simulink model "afe_inv_ttype_psm"  (R2026a)
settings: Solver=ode23tb  StopTime=simlength  FixedStep=tc  MaxStep=glb_time.tc
values from neighbouring files (symbols this model uses):
  afe_ctrl = ctrl_afe_setup(glb_time.ts_afe, grid_emu.omega_grid_nom)    [init_model.m]
  afe_pwm_phase_shift_mod1 = 0    [init_model.m]
  DThs_init = 0    [init_model.m]
  filters = setup_global_filters(glb_time.ts_afe, glb_time.ts_inv, glb_time.ts_dab, glb_time.tc)    [init_model.m]
  frt_data = frt_settings(test_index, test_subindex, asymmetric_error_type,      enable_frt_1, enable_frt_2, start_time_LVRT, deepPOSxi, deepPOSeta, deepNEGxi, deepNEGeta)    [init_model.m]
  glb_time = timing_setup(fpwm_afe, trgo_afe, fpwm_inv, trgo_inv, fpwm_single_phase_inv, trgo_single_phase_inv, fpwm_dab, trgo_dab,      fpwm_psfbc, trgo_psfbc, fpwm_isop_rail, trgo_isop_rail, fpwm_cllc, trgo_cllc, t_measure, tc_factor, tc_decimation, delay_pwm, dead_time_afe,      dead_time_inv, dead_time_single_phase_inv, dead_time_dab, dead_time_psfbc, dead_time_isop_rail, dead_time_cllc)    [init_model.m]
  grid_emu = grid_three_phase_emulator('Dyn11', delta_star, grid_nominal_power, application_voltage, us1, us2, fgrid,                  eq_grid_inductance, eq_grid_resistance, eta, ucc, i1m, p_iron, n1, n2, core_area, core_length, mur,                  up_xi_pu_ref, up_eta_pu_ref, un_xi_pu_ref, un_eta_pu_ref)    [init_model.m]
  i_react_pos_ref_2 = -ixi_ref_mod1*tan(acos(0.95))    [init_model.m]
  i_react_pos_ref_3 = ixi_ref_mod1*tan(acos(0.95))    [init_model.m]
  ixi_ref_mod1 = -0.85    [init_model.m]
  ki_align = 18    [init_model.m]
  kp_align = 0.25    [init_model.m]
  lim_down_align = -0.05    [init_model.m]
  lim_up_align = 0.05    [init_model.m]
  mavarage_filter_frequency_base_order = 2    [init_model.m]
  omega_m_sim = psm.omega_m_bez    [init_model.m]
  psm = psm_calculus()    [init_model.m]
  psm_ctrl = ctrl_pmsm_setup(glb_time.ts_inv, psm.omega_bez, u_psm_scale, psm.Jm_norm)    [init_model.m]
  simlength = 1.75    [init_model.m]
  Tambient = 40    [init_model.m]
  time_aux_power_supply_fault = 1e3    (= 1000)    [init_model.m]
  time_gain_afe_module_1 = 1.0002    [init_model.m]
  time_gain_inv_module_2 = 1.001    [init_model.m]
  time_i_react_pos_ref_1 = start_time_LVRT + error_length + 0.335    [init_model.m]
  time_i_react_pos_ref_2 = time_i_react_pos_ref_1 + 0.5    (= 0.5)    [init_model.m]
  time_start_motor_control = 0.25    [init_model.m]
  torque_overload_factor = 1    [init_model.m]
  u_cm_comp_mod1 = 0    [init_model.m]
  u_psm_scale_ekf = sqrt(3)/2 * 2/3 * hwdata.inv.udc_nom/psm.ubez    [init_model.m]
undefined symbols (not defined in the file or in its folder): hwdata, magnitude, omega_m_bez, rpm_base, torque_base
libraries: fl_lib x74, nesl_utility x43, moving_average_filter x10, moving_average_filter_cc x8, discrete_time_low_pass_filter x4, sl_discontinuities x3, single_phase_transformer_lib x3, linear_double_integrator_observer_ccaller x2, threephase_inductor_lib x2, dclink_for_three_levels x2, three_phase_three_level_ttype_inverter_ideal_switch_based_model x2, cstblocks_lti x2
(part 2 of 9)

== system afe_inv_ttype_psm/global timing/time_afe3 ==
  Gain : Gain  Gain=k
  time_1 : Clock
  Out1 : Outport
  wires:
  Gain/1 -> Out1/1
  time_1/1 -> Gain/1

== system afe_inv_ttype_psm/global timing/time_inv1 ==
  correction_time : Inport
  Constant : Constant
  Gain : Gain  Gain=k
  Product : Product
  Sum : Sum  Inputs=|++
  time_1 : Clock
  Out1 : Outport
  wires:
  time_1/1 -> Gain/1
  Gain/1 -> Product/1
  Product/1 -> Out1/1
  correction_time/1 -> Sum/1
  Constant/1 -> Sum/2
  Sum/1 -> Product/2

== system afe_inv_ttype_psm/grid/grid_emulator ==
  3ph_Dyg : Subsystem
  Bus Selector : BusSelector  OutputSignals=ua_grid_emu,ub_grid_emu,uc_grid_emu
  Bus Selector1 : BusSelector  OutputSignals=gamma_grid_emulator,omega_grid_emulator
  Controlled Voltage Source : fl_lib/Electrical/Electrical Sources/Controlled Voltage Source
  Controlled Voltage Source1 : fl_lib/Electrical/Electrical Sources/Controlled Voltage Source
  Controlled Voltage Source2 : fl_lib/Electrical/Electrical Sources/Controlled Voltage Source
  Electrical Reference : fl_lib/Electrical/Electrical Elements/Electrical Reference
  Simulink-PS Converter : nesl_utility/Simulink-PS Converter  PhysicalDomain=network_engine_domain  SubClassName=ps_input  LeftPortType=input  RightPortType=output  PseudoPeriodic=off  Frequencies=[]  NoiseDistribution=none  NoiseParameters=[]  Unit=V  AffineConversion=on  FilteringAndDerivatives=provide  SimscapeFilterOrder=1  InputFilterTimeConstant=0.001  UdotUserProvided=0
  Simulink-PS Converter1 : nesl_utility/Simulink-PS Converter  PhysicalDomain=network_engine_domain  SubClassName=ps_input  LeftPortType=input  RightPortType=output  PseudoPeriodic=off  Frequencies=[]  NoiseDistribution=none  NoiseParameters=[]  Unit=V  AffineConversion=on  FilteringAndDerivatives=provide  SimscapeFilterOrder=1  InputFilterTimeConstant=0.001  UdotUserProvided=0
  Simulink-PS Converter2 : nesl_utility/Simulink-PS Converter  PhysicalDomain=network_engine_domain  SubClassName=ps_input  LeftPortType=input  RightPortType=output  PseudoPeriodic=off  Frequencies=[]  NoiseDistribution=none  NoiseParameters=[]  Unit=V  AffineConversion=on  FilteringAndDerivatives=provide  SimscapeFilterOrder=1  InputFilterTimeConstant=0.001  UdotUserProvided=0
  Solver Configuration : nesl_utility/Solver Configuration  PhysicalDomain=network_engine_domain  SubClassName=solver  LeftPortType=input  RightPortType=generic  Tones=[]  Harmonics=[]  SimulateNoise=off  Profile=off  UseLocalSampling=off  EnableSwitchedLinearOptims=on  FrequencyDomain=off  UseCCode=off  RelTol=0.001  AbsTol=0.001  MinStep=1e-09  ToWorkspace=off  RevertToSquareIcSolve=off  NumHomotopyIterations=100  PhasorMode=off  PhasorModeNumHarmonics=1  ConsistencySolver=NEWTON_FTOL  CanonicalOrdering=UNORDERED  OptimizeIntermediates=UNOPTIMIZED  IndexReductionMethod=DerivativeReplacement  DoDC=on  ResidualTolerance=1e-09  ConsistencyTolSource=GLOBAL  ConsistencyAbsTol=0.001  ConsistencyRelTol=0.001  ConsistencyTolFactor=0.001  UseLocalSolver=on  LocalSolverChoice=NE_BACKWARD_EULER_ADVANCER  ResolveIndetEquations=on  FunctionEvalNumThread=1  LocalSolverSampleTime=glb_time.tc  DoFixedCost=on  MaxNonlinIter=nonlinear_iterations  MaxModeIter=2  ComputeImpulses=off  ImpulseIterations=2  LinearAlgebra=auto  LinearAlgebraNumThread=0  EquationFormulation=NE_TIME_EF  DelaysMemoryBudget=1024  AutomaticFiltering=on  FilteringTimeConstant=0.001  PartitionStorageMethod=AS_NEEDED  PartitionMemoryBudget=1024  PartitionMethod=ROBUST  MultibodyUseLocalSolver=off  MultibodyLocalSolverChoice=ODE1  MultibodyLocalSolverSampleTime=0.001
  three_phase_voltage_source_with_frt_emulator : three_phase_voltage_with_frt_emulator/three_phase_voltage_source_with_frt_emulator  nominal_frequency_m=grid_emu.fgrid_nom  nominal_voltage_m=grid_emu.us_primary_nom  Vemu_ref_norm_m=grid_emu.Vemu_ref_norm  vp_xi_pu_m=grid_emu.up_xi_pu_ref  vp_eta_pu_m=grid_emu.up_eta_pu_ref  vn_xi_pu_m=grid_emu.un_xi_pu_ref  vn_eta_pu_m=grid_emu.un_eta_pu_ref  Am=filters.afe.SOF_50Hz.ss_c.A  Bm=filters.afe.SOF_50Hz.ss_c.B  Cm=filters.afe.SOF_50Hz.ss_c.C  enable_frt_1_m=frt_data.enable_frt_1  enable_frt_2_m=frt_data.enable_frt_2  start_time_LVRT_m=frt_data.start_time_LVRT  end_time_LVRT_m=frt_data.end_time_LVRT  deepPOSxi_m=frt_data.deepPOSxi  deepPOSeta_m=frt_data.deepPOSeta  deepNEGxi_m=frt_data.deepNEGxi  deepNEGeta_m=frt_data.deepNEGeta  Amplitude_U_m=frt_data.Amplitude_U  Amplitude_V_m=frt_data.Amplitude_V  Amplitude_W_m=frt_data.Amplitude_W  t_ramp_m=frt_data.t_ramp  Phase_shift_m=frt_data.Phase_shift
  threephase_vi_measures : Subsystem
  u1 : PMIOPort  Side=Right
  u2 : PMIOPort  Port=2  Side=Right
  u3 : PMIOPort  Port=3  Side=Right
  tag scope: gamma_grid_emulator=global, omega_grid_emulator=global
  wires:
  Bus Selector1/2 -> [omega_grid_emulator]  "<omega_grid_emulator>"
  Bus Selector1/1 -> [gamma_grid_emulator]  "<gamma_grid_emulator>"
  Bus Selector/2 -> Simulink-PS Converter1/1  "<ub_grid_emu>"
  Bus Selector/3 -> Simulink-PS Converter2/1  "<uc_grid_emu>"
  three_phase_voltage_source_with_frt_emulator/1 -> Bus Selector1/1, Bus Selector/1
  Bus Selector/1 -> Simulink-PS Converter/1  "<ua_grid_emu>"
  connections:
  Simulink-PS Converter/RConn1 -- Controlled Voltage Source/RConn1
  Simulink-PS Converter1/RConn1 -- Controlled Voltage Source1/RConn1
  Simulink-PS Converter2/RConn1 -- Controlled Voltage Source2/RConn1
  Electrical Reference/LConn1 -- Controlled Voltage Source/RConn2 -- Controlled Voltage Source1/RConn2 -- Controlled Voltage Source2/RConn2 -- Solver Configuration/RConn1
  3ph_Dyg/RConn1 -- u1/RConn1
  3ph_Dyg/RConn2 -- u2/RConn1
  3ph_Dyg/RConn3 -- u3/RConn1
  3ph_Dyg/LConn1 -- threephase_vi_measures/RConn1
  3ph_Dyg/LConn2 -- threephase_vi_measures/RConn2
  3ph_Dyg/LConn3 -- threephase_vi_measures/RConn3
  Controlled Voltage Source/LConn1 -- threephase_vi_measures/LConn1
  Controlled Voltage Source1/LConn1 -- threephase_vi_measures/LConn2
  Controlled Voltage Source2/LConn1 -- threephase_vi_measures/LConn3

== system afe_inv_ttype_psm/grid/threephase_vi_measures ==
  Bus Creator : BusCreator  Inputs=6
  Current Sensor : fl_lib/Electrical/Electrical Sensors/Current Sensor
  Current Sensor1 : fl_lib/Electrical/Electrical Sensors/Current Sensor
  Current Sensor2 : fl_lib/Electrical/Electrical Sensors/Current Sensor
  Electrical Reference1 : fl_lib/Electrical/Electrical Elements/Electrical Reference
  Selector : Selector  InputPortWidth=6  IndexOptions=Index vector (dialog)  Indices=[1 2 3]  OutputSizes=1
  Selector1 : Selector  InputPortWidth=6  IndexOptions=Index vector (dialog)  Indices=[4 5 6]  OutputSizes=1
  Voltage Sensor : fl_lib/Electrical/Electrical Sensors/Voltage Sensor
  Voltage Sensor1 : fl_lib/Electrical/Electrical Sensors/Voltage Sensor
  Voltage Sensor2 : fl_lib/Electrical/Electrical Sensors/Voltage Sensor
  ia_grid : nesl_utility/PS-Simulink Converter  PhysicalDomain=network_engine_domain  SubClassName=ps_output  LeftPortType=input  RightPortType=output  PseudoPeriodic=off  Frequencies=[]  VectorFormat=1-D array  Unit=A  AffineConversion=off
  ib_grid : nesl_utility/PS-Simulink Converter  PhysicalDomain=network_engine_domain  SubClassName=ps_output  LeftPortType=input  RightPortType=output  PseudoPeriodic=off  Frequencies=[]  VectorFormat=1-D array  Unit=A  AffineConversion=off
  ic_grid : nesl_utility/PS-Simulink Converter  PhysicalDomain=network_engine_domain  SubClassName=ps_output  LeftPortType=input  RightPortType=output  PseudoPeriodic=off  Frequencies=[]  VectorFormat=1-D array  Unit=A  AffineConversion=off
  ig_abc/ug_abc : Scope  NumInputPorts=2
      settings: SampleTime=glb_time.tc  ActiveDisplayYMinimum=-662.618491750231  ActiveDisplayYMaximum=662.00821995187164  DataLoggingVariableName=ScopeData2
  ua_grid : nesl_utility/PS-Simulink Converter  PhysicalDomain=network_engine_domain  SubClassName=ps_output  LeftPortType=input  RightPortType=output  PseudoPeriodic=off  Frequencies=[]  VectorFormat=1-D array  Unit=V  AffineConversion=off
  ub_grid : nesl_utility/PS-Simulink Converter  PhysicalDomain=network_engine_domain  SubClassName=ps_output  LeftPortType=input  RightPortType=output  PseudoPeriodic=off  Frequencies=[]  VectorFormat=1-D array  Unit=V  AffineConversion=off
  uc_grid : nesl_utility/PS-Simulink Converter  PhysicalDomain=network_engine_domain  SubClassName=ps_output  LeftPortType=input  RightPortType=output  PseudoPeriodic=off  Frequencies=[]  VectorFormat=1-D array  Unit=V  AffineConversion=off
  Ua : PMIOPort  Side=Left
  ua : PMIOPort  Port=2  Side=Right
  Ub : PMIOPort  Port=3  Side=Left
  ub : PMIOPort  Port=4  Side=Right
  Uc : PMIOPort  Port=5  Side=Left
  uc : PMIOPort  Port=6  Side=Right
  tag scope: ig_abc=global, ug_abc=global
  wires:
  Bus Creator/1 -> Selector1/1, Selector/1  "vi_data"
  Selector/1 -> [ug_abc]
  ib_grid/1 -> Bus Creator/5  "ib"
  ia_grid/1 -> Bus Creator/4  "ia"
  ic_grid/1 -> Bus Creator/6  "ic"
  ua_grid/1 -> Bus Creator/1  "ua"
  ub_grid/1 -> Bus Creator/2  "ub"
  uc_grid/1 -> Bus Creator/3  "uc"
  Selector1/1 -> [ig_abc]
  [ug_abc] -> ig_abc/ug_abc/2  "ug_abc(line)"
  [ig_abc] -> ig_abc/ug_abc/1  "ig_abc(line)"
  connections:
  Current Sensor1/LConn1 -- Ub/RConn1 -- Voltage Sensor1/LConn1
  Electrical Reference1/LConn1 -- Voltage Sensor/RConn2 -- Voltage Sensor2/RConn2 -- Voltage Sensor1/RConn2
  Voltage Sensor/RConn1 -- ua_grid/LConn1
  Current Sensor/RConn2 -- ua/RConn1
  Voltage Sensor1/RConn1 -- ub_grid/LConn1
  Voltage Sensor2/LConn1 -- Current Sensor2/LConn1 -- Uc/RConn1
  Current Sensor/LConn1 -- Ua/RConn1 -- Voltage Sensor/LConn1
  Current Sensor1/RConn2 -- ub/RConn1
  Voltage Sensor2/RConn1 -- uc_grid/LConn1
  ib_grid/LConn1 -- Current Sensor1/RConn1
  ia_grid/LConn1 -- Current Sensor/RConn1
  ic_grid/LConn1 -- Current Sensor2/RConn1
  Current Sensor2/RConn2 -- uc/RConn1

== system afe_inv_ttype_psm/inverter_measurement_sim/module_1 ==
  To Workspace12 : ToWorkspace  VariableName=ileg_dc_inv_sim_mod1  SampleTime=glb_time.tc
      settings: MaxDataPoints=glb_time.Nc
  To Workspace14 : ToWorkspace  VariableName=is_uvw_sim_mod1  SampleTime=glb_time.tc
      settings: MaxDataPoints=glb_time.Nc
  To Workspace15 : ToWorkspace  VariableName=us_uvw_sim_mod1  SampleTime=glb_time.tc
      settings: MaxDataPoints=glb_time.Nc
  wires:
  [us_uvw_pu_mod1] -> To Workspace15/1
  [ileg_dc_inv_mod1] -> To Workspace12/1
  [is_uvw_pu_mod1] -> To Workspace14/1

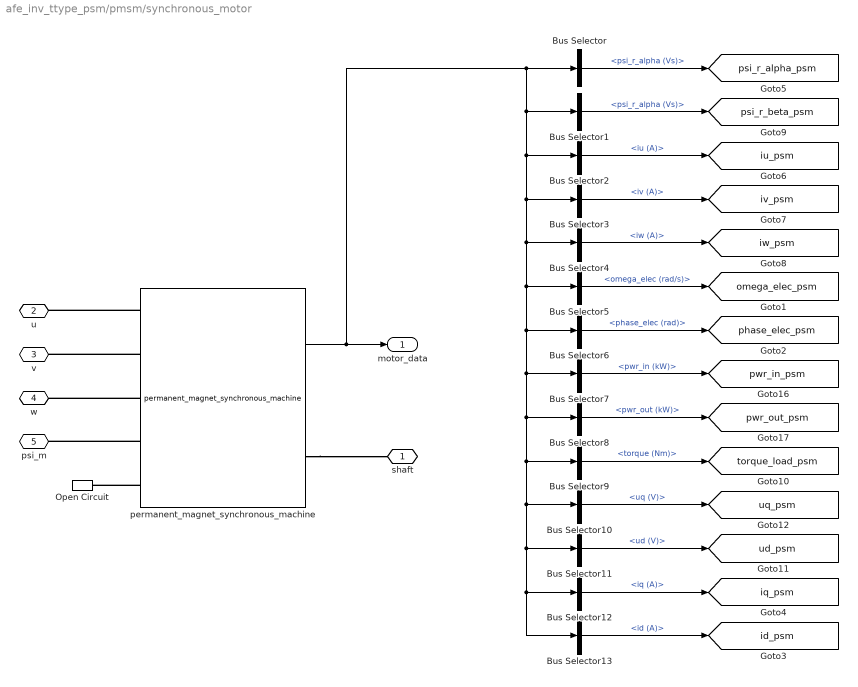
== system afe_inv_ttype_psm/pmsm/synchronous_motor ==
  Bus Selector : BusSelector  OutputSignals=psi_r_alpha (Vs)
  Bus Selector1 : BusSelector  OutputSignals=psi_r_alpha (Vs)
  Bus Selector10 : BusSelector  OutputSignals=uq (V)
  Bus Selector11 : BusSelector  OutputSignals=ud (V)
  Bus Selector12 : BusSelector  OutputSignals=iq (A)
  Bus Selector13 : BusSelector  OutputSignals=id (A)
  Bus Selector2 : BusSelector  OutputSignals=iu (A)
  Bus Selector3 : BusSelector  OutputSignals=iv (A)
  Bus Selector4 : BusSelector  OutputSignals=iw (A)
  Bus Selector5 : BusSelector  OutputSignals=omega_elec (rad/s)
  Bus Selector6 : BusSelector  OutputSignals=phase_elec (rad)
  Bus Selector7 : BusSelector  OutputSignals=pwr_in (kW)
  Bus Selector8 : BusSelector  OutputSignals=pwr_out (kW)
  Bus Selector9 : BusSelector  OutputSignals=torque (Nm)
  Open Circuit : fl_lib/Electrical/Electrical Elements/Open Circuit  v_specify=off  v_priority=None  v=0 V  v_nominal_specify=off  v_nominal_value=1  v_nominal_unit=V
  permanent_magnet_synchronous_machine : permanent_magnet_synchronous_machine/permanent_magnet_synchronous_machine  pp=psm.number_poles  psi_m=psm.psi_m  Lmu=psm.Lmu  La=psm.La_m  Lb=psm.Lb_m  Rs=psm.Rs_m  Jm=psm.Jm_m  b_linear=psm.load_friction_m  b_quadratic=0  h5_percent=0  h7_percent=0  psi_r_u_init=psm.psi_m  psi_r_v_init=-psm.psi_m/2  psi_r_w_init=-psm.psi_m/2  omega_init=0  phase_init=0
  shaft : PMIOPort  Side=Right
  u : PMIOPort  Port=2  Side=Left
  v : PMIOPort  Port=3  Side=Left
  w : PMIOPort  Port=4  Side=Left
  psi_m : PMIOPort  Port=5  Side=Left
  motor_data : Outport
  tag scope: id_psm=global, iq_psm=global, iu_psm=global, iv_psm=global, iw_psm=global, omega_elec_psm=global, phase_elec_psm=global, psi_r_alpha_psm=global, psi_r_beta_psm=global, pwr_in_psm=global, pwr_out_psm=global, torque_load_psm=global, ud_psm=global, uq_psm=global
  wires:
  permanent_magnet_synchronous_machine/1 -> Bus Selector8/1, Bus Selector10/1, Bus Selector11/1, Bus Selector12/1, Bus Selector13/1, Bus Selector9/1, Bus Selector7/1, Bus Selector6/1, Bus Selector5/1, Bus Selector4/1, Bus Selector3/1, Bus Selector2/1, Bus Selector1/1, Bus Selector/1, motor_data/1
  Bus Selector/1 -> [psi_r_alpha_psm]  "<psi_r_alpha (Vs)>"
  Bus Selector1/1 -> [psi_r_beta_psm]  "<psi_r_alpha (Vs)>"
  Bus Selector2/1 -> [iu_psm]  "<iu (A)>"
  Bus Selector3/1 -> [iv_psm]  "<iv (A)>"
  Bus Selector4/1 -> [iw_psm]  "<iw (A)>"
  Bus Selector5/1 -> [omega_elec_psm]  "<omega_elec (rad/s)>"
  Bus Selector6/1 -> [phase_elec_psm]  "<phase_elec (rad)>"
  Bus Selector7/1 -> [pwr_in_psm]  "<pwr_in (kW)>"
  Bus Selector8/1 -> [pwr_out_psm]  "<pwr_out (kW)>"
  Bus Selector9/1 -> [torque_load_psm]  "<torque (Nm)>"
  Bus Selector10/1 -> [uq_psm]  "<uq (V)>"
  Bus Selector11/1 -> [ud_psm]  "<ud (V)>"
  Bus Selector12/1 -> [iq_psm]  "<iq (A)>"
  Bus Selector13/1 -> [id_psm]  "<id (A)>"
  connections:
  permanent_magnet_synchronous_machine/RConn1 -- shaft/RConn1
  permanent_magnet_synchronous_machine/LConn1 -- u/RConn1
  permanent_magnet_synchronous_machine/LConn2 -- v/RConn1
  permanent_magnet_synchronous_machine/LConn3 -- w/RConn1
  permanent_magnet_synchronous_machine/LConn4 -- psi_m/RConn1
  permanent_magnet_synchronous_machine/LConn5 -- Open Circuit/LConn1

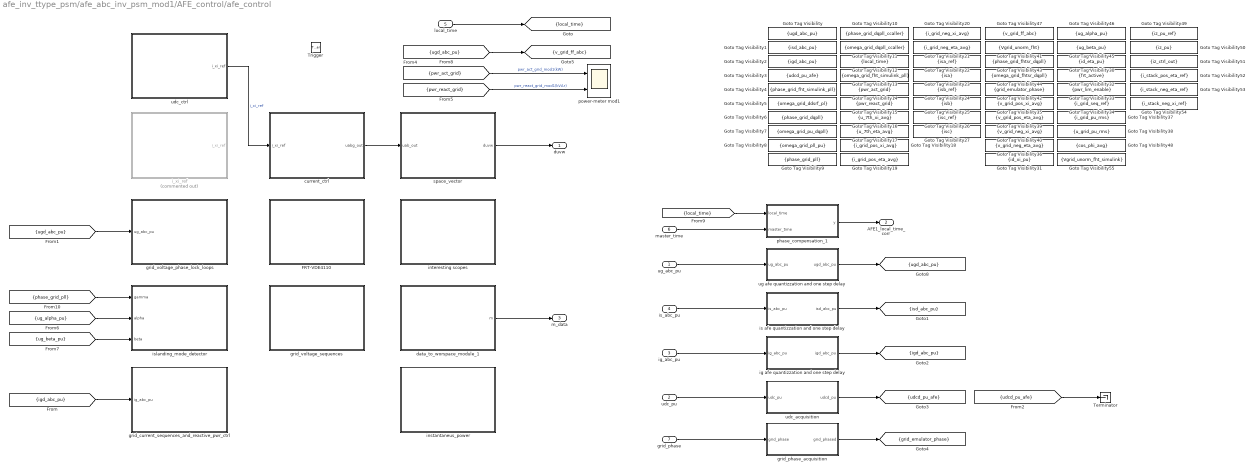
== system afe_inv_ttype_psm/afe_abc_inv_psm_mod1/AFE_control/afe_control ==
  ug_abc_pu : Inport
  udc_pu : Inport  Port=2
  ig_abc_pu : Inport  Port=3
  is_abc_pu : Inport  Port=4
  local_time : Inport  Port=5
  master_time : Inport  Port=6
  grid_phase : Inport  Port=7
  Trigger : TriggerPort  VariantControl=(inherit)  PortDimensions=1
  FRT-VDE4110 : Subsystem
  Goto Tag Visibility : GotoTagVisibility  GotoTag=ugd_abc_pu
  Goto Tag Visibility1 : GotoTagVisibility  GotoTag=isd_abc_pu
  Goto Tag Visibility10 : GotoTagVisibility  GotoTag=phase_grid_dqpll_ccaller
  Goto Tag Visibility11 : GotoTagVisibility  GotoTag=omega_grid_dqpll_ccaller
  Goto Tag Visibility12 : GotoTagVisibility  GotoTag=local_time
  Goto Tag Visibility13 : GotoTagVisibility  GotoTag=omega_grid_fht_simulink_pll
  Goto Tag Visibility14 : GotoTagVisibility  GotoTag=pwr_act_grid
  Goto Tag Visibility15 : GotoTagVisibility  GotoTag=pwr_react_grid
  Goto Tag Visibility16 : GotoTagVisibility  GotoTag=u_7th_xi_avg
  Goto Tag Visibility17 : GotoTagVisibility  GotoTag=u_7th_eta_avg
  Goto Tag Visibility18 : GotoTagVisibility  GotoTag=i_grid_pos_xi_avg
  Goto Tag Visibility19 : GotoTagVisibility  GotoTag=i_grid_pos_eta_avg
  Goto Tag Visibility2 : GotoTagVisibility  GotoTag=igd_abc_pu
  Goto Tag Visibility20 : GotoTagVisibility  GotoTag=i_grid_neg_xi_avg
  Goto Tag Visibility21 : GotoTagVisibility  GotoTag=i_grid_neg_eta_avg
  Goto Tag Visibility22 : GotoTagVisibility  GotoTag=isa_ref
  Goto Tag Visibility23 : GotoTagVisibility  GotoTag=isa
  Goto Tag Visibility24 : GotoTagVisibility  GotoTag=isb_ref
  Goto Tag Visibility25 : GotoTagVisibility  GotoTag=isb
  Goto Tag Visibility26 : GotoTagVisibility  GotoTag=isc_ref
  Goto Tag Visibility27 : GotoTagVisibility  GotoTag=isc
  Goto Tag Visibility3 : GotoTagVisibility  GotoTag=udcd_pu_afe
  Goto Tag Visibility30 : GotoTagVisibility  GotoTag=id_eta_pu
  Goto Tag Visibility31 : GotoTagVisibility  GotoTag=id_xi_pu
  Goto Tag Visibility32 : GotoTagVisibility  GotoTag=frt_active
  Goto Tag Visibility33 : GotoTagVisibility  GotoTag=pwr_lim_enable
  Goto Tag Visibility34 : GotoTagVisibility  GotoTag=i_grid_seq_ref
  Goto Tag Visibility35 : GotoTagVisibility  GotoTag=v_grid_pos_xi_avg
  Goto Tag Visibility36 : GotoTagVisibility  GotoTag=v_grid_neg_eta_avg
  Goto Tag Visibility37 : GotoTagVisibility  GotoTag=i_grid_pu_rms
  Goto Tag Visibility38 : GotoTagVisibility  GotoTag=u_grid_pu_rms
  Goto Tag Visibility39 : GotoTagVisibility  GotoTag=v_grid_pos_eta_avg
  Goto Tag Visibility4 : GotoTagVisibility  GotoTag=phase_grid_fht_simulink_pll
  Goto Tag Visibility40 : GotoTagVisibility  GotoTag=v_grid_neg_xi_avg
  Goto Tag Visibility41 : GotoTagVisibility  GotoTag=Vgrid_unorm_fht
  Goto Tag Visibility42 : GotoTagVisibility  GotoTag=grid_emulator_phase
  Goto Tag Visibility43 : GotoTagVisibility  GotoTag=phase_grid_fhtsr_dqpll
  Goto Tag Visibility44 : GotoTagVisibility  GotoTag=omega_grid_fhtsr_dqpll
  Goto Tag Visibility45 : GotoTagVisibility  GotoTag=ug_beta_pu
  Goto Tag Visibility46 : GotoTagVisibility  GotoTag=ug_alpha_pu
  Goto Tag Visibility47 : GotoTagVisibility  GotoTag=v_grid_ff_abc
  Goto Tag Visibility48 : GotoTagVisibility  GotoTag=cos_phi_avg
  Goto Tag Visibility49 : GotoTagVisibility  GotoTag=iz_pu_ref
  Goto Tag Visibility5 : GotoTagVisibility  GotoTag=omega_grid_ddsrf_pl
  Goto Tag Visibility50 : GotoTagVisibility  GotoTag=iz_pu
  Goto Tag Visibility51 : GotoTagVisibility  GotoTag=iz_ctrl_out
  Goto Tag Visibility52 : GotoTagVisibility  GotoTag=i_stack_pos_eta_ref
  Goto Tag Visibility53 : GotoTagVisibility  GotoTag=i_stack_neg_eta_ref
  Goto Tag Visibility54 : GotoTagVisibility  GotoTag=i_stack_neg_xi_ref
  Goto Tag Visibility55 : GotoTagVisibility  GotoTag=Vgrid_unorm_fht_simulink
  Goto Tag Visibility6 : GotoTagVisibility  GotoTag=phase_grid_dqpll
  Goto Tag Visibility7 : GotoTagVisibility  GotoTag=omega_grid_pu_dqpll
  Goto Tag Visibility8 : GotoTagVisibility  GotoTag=omega_grid_pll_pu
  Goto Tag Visibility9 : GotoTagVisibility  GotoTag=phase_grid_pll
  Terminator : Terminator
  current_ctrl : Subsystem
  data_to_worspace_module_1 : Subsystem
  grid_current_sequences_and_reactive_pwr_ctrl : Subsystem
  grid_phase_acquisition : Subsystem
  grid_voltage_phase_lock_loops : Subsystem
  grid_voltage_sequences : Subsystem
  i_xi_ref : Subsystem  Commented=on
  ig afe quantizzation and one step delay : Subsystem
  instantaneus_power : Subsystem
  interesting scopes : Subsystem
  is afe quantizzation and one step delay : Subsystem
  islanding_mode_detector : Subsystem
  phase_compensation_1 : Subsystem
  power-meter mod1 : Scope  NumInputPorts=2
      settings: ActiveDisplayYMinimum=-271.22706700611354  ActiveDisplayYMaximum=172.30597192664806  DataLoggingVariableName=ScopeData9
  space_vector : Subsystem
  udc_acquisition : Subsystem
  udc_ctrl : Subsystem
  ug afe quantizzation and one step delay : Subsystem
  duvw : Outport
  AFE1_local_time_corr : Outport  Port=2
  m_data : Outport  Port=3
  tag scope: grid_emulator_phase=scoped, igd_abc_pu=scoped, isd_abc_pu=scoped, local_time=scoped, udcd_pu_afe=scoped, ugd_abc_pu=scoped, v_grid_ff_abc=scoped
  wires:
  ug_abc_pu/1 -> ug afe quantizzation and one step delay/1(ug_abc_pu)
  current_ctrl/1(uabg_out) -> space_vector/1(uab_out)
  space_vector/1(duvw) -> duvw/1
  is_abc_pu/1 -> is afe quantizzation and one step delay/1(is_abc_pu)
  ig_abc_pu/1 -> ig afe quantizzation and one step delay/1(ig_abc_pu)
  [ugd_abc_pu] -> grid_voltage_phase_lock_loops/1(ug_abc_pu)
  [igd_abc_pu] -> grid_current_sequences_and_reactive_pwr_ctrl/1(ig_abc_pu)
  udc_pu/1 -> udc_acquisition/1(udc_pu)
  udc_acquisition/1(udcd_pu) -> [udcd_pu_afe]
  [pwr_react_grid] -> power-meter mod1/2  "pwr_react_grid_mod1(kVAr)"
  [pwr_act_grid] -> power-meter mod1/1  "pwr_act_grid_mod1(kW)"
  [phase_grid_pll] -> islanding_mode_detector/1(gamma)
  [ug_alpha_pu] -> islanding_mode_detector/2(alpha)
  ug afe quantizzation and one step delay/1(ugd_abc_pu) -> [ugd_abc_pu]
  is afe quantizzation and one step delay/1(isd_abc_pu) -> [isd_abc_pu]
  ig afe quantizzation and one step delay/1(igd_abc_pu) -> [igd_abc_pu]
  [ug_beta_pu] -> islanding_mode_detector/3(beta)
  local_time/1 -> [local_time]
  master_time/1 -> phase_compensation_1/2(master_time)
  phase_compensation_1/1(y) -> AFE1_local_time_corr/1
  [local_time] -> phase_compensation_1/1(local_time)
  grid_phase/1 -> grid_phase_acquisition/1(grid_phase)
  grid_phase_acquisition/1(grid_phased) -> [grid_emulator_phase]
  [ugd_abc_pu] -> [v_grid_ff_abc]
  data_to_worspace_module_1/1(m) -> m_data/1
  [udcd_pu_afe] -> Terminator/1
  udc_ctrl/1(i_xi_ref) -> current_ctrl/1(i_xi_ref)  "i_xi_ref"

== system afe_inv_ttype_psm/afe_abc_inv_psm_mod1/LCL_filter/threephase_vi_measures_grid ==
  Bus Creator : BusCreator  Inputs=6
  Current Sensor : fl_lib/Electrical/Electrical Sensors/Current Sensor
  Current Sensor1 : fl_lib/Electrical/Electrical Sensors/Current Sensor
  Current Sensor2 : fl_lib/Electrical/Electrical Sensors/Current Sensor
  Electrical Reference1 : fl_lib/Electrical/Electrical Elements/Electrical Reference
  Gain1 : Gain  Gain=1/hwdata.afe.ubez
  Gain2 : Gain  Gain=1/hwdata.afe.ubez
  Gain3 : Gain  Gain=1/hwdata.afe.ubez
  Gain4 : Gain  Gain=1/hwdata.afe.ibez
  Gain5 : Gain  Gain=1/hwdata.afe.ibez
  Gain6 : Gain  Gain=1/hwdata.afe.ibez
  Selector : Selector  InputPortWidth=6  IndexOptions=Index vector (dialog)  Indices=[1 2 3]  OutputSizes=1
  Selector1 : Selector  InputPortWidth=6  IndexOptions=Index vector (dialog)  Indices=[4 5 6]  OutputSizes=1
  Voltage Sensor : fl_lib/Electrical/Electrical Sensors/Voltage Sensor
  Voltage Sensor1 : fl_lib/Electrical/Electrical Sensors/Voltage Sensor
  Voltage Sensor2 : fl_lib/Electrical/Electrical Sensors/Voltage Sensor
  ia_grid : nesl_utility/PS-Simulink Converter  PhysicalDomain=network_engine_domain  SubClassName=ps_output  LeftPortType=input  RightPortType=output  PseudoPeriodic=off  Frequencies=[]  VectorFormat=1-D array  Unit=A  AffineConversion=off
  ib_grid : nesl_utility/PS-Simulink Converter  PhysicalDomain=network_engine_domain  SubClassName=ps_output  LeftPortType=input  RightPortType=output  PseudoPeriodic=off  Frequencies=[]  VectorFormat=1-D array  Unit=A  AffineConversion=off
  ic_grid : nesl_utility/PS-Simulink Converter  PhysicalDomain=network_engine_domain  SubClassName=ps_output  LeftPortType=input  RightPortType=output  PseudoPeriodic=off  Frequencies=[]  VectorFormat=1-D array  Unit=A  AffineConversion=off
  ua_grid : nesl_utility/PS-Simulink Converter  PhysicalDomain=network_engine_domain  SubClassName=ps_output  LeftPortType=input  RightPortType=output  PseudoPeriodic=off  Frequencies=[]  VectorFormat=1-D array  Unit=V  AffineConversion=off
  ub_grid : nesl_utility/PS-Simulink Converter  PhysicalDomain=network_engine_domain  SubClassName=ps_output  LeftPortType=input  RightPortType=output  PseudoPeriodic=off  Frequencies=[]  VectorFormat=1-D array  Unit=V  AffineConversion=off
  uc_grid : nesl_utility/PS-Simulink Converter  PhysicalDomain=network_engine_domain  SubClassName=ps_output  LeftPortType=input  RightPortType=output  PseudoPeriodic=off  Frequencies=[]  VectorFormat=1-D array  Unit=V  AffineConversion=off
  Ua : PMIOPort  Side=Left
  ua : PMIOPort  Port=2  Side=Right
  Ub : PMIOPort  Port=3  Side=Left
  ub : PMIOPort  Port=4  Side=Right
  Uc : PMIOPort  Port=5  Side=Left
  uc : PMIOPort  Port=6  Side=Right
  tag scope: ig_abc_pu_mod1=global, ug_abc_pu_mod1=global
  wires:
  Selector1/1 -> [ig_abc_pu_mod1]
  uc_grid/1 -> Gain3/1
  ub_grid/1 -> Gain2/1
  ua_grid/1 -> Gain1/1
  ic_grid/1 -> Gain5/1
  ia_grid/1 -> Gain6/1
  ib_grid/1 -> Gain4/1
  Selector/1 -> [ug_abc_pu_mod1]
  Bus Creator/1 -> Selector1/1, Selector/1  "vi_data"
  Gain1/1 -> Bus Creator/1  "ua_grid_pu"
  Gain2/1 -> Bus Creator/2  "ub_grid_pu"
  Gain3/1 -> Bus Creator/3  "uc_grid_pu"
  Gain6/1 -> Bus Creator/4  "ia_grid_pu"
  Gain4/1 -> Bus Creator/5  "ib_grid_pu"
  Gain5/1 -> Bus Creator/6  "ic_grid_pu"
  connections:
  Current Sensor2/RConn2 -- uc/RConn1
  ic_grid/LConn1 -- Current Sensor2/RConn1
  ia_grid/LConn1 -- Current Sensor/RConn1
  ib_grid/LConn1 -- Current Sensor1/RConn1
  Voltage Sensor2/RConn1 -- uc_grid/LConn1
  Current Sensor1/RConn2 -- ub/RConn1
  Voltage Sensor/LConn1 -- Current Sensor/LConn1 -- Ua/RConn1
  Current Sensor2/LConn1 -- Voltage Sensor2/LConn1 -- Uc/RConn1
  Voltage Sensor1/RConn1 -- ub_grid/LConn1
  Current Sensor/RConn2 -- ua/RConn1
  Voltage Sensor/RConn1 -- ua_grid/LConn1
  Voltage Sensor1/RConn2 -- Voltage Sensor2/RConn2 -- Voltage Sensor/RConn2 -- Electrical Reference1/LConn1
  Voltage Sensor1/LConn1 -- Current Sensor1/LConn1 -- Ub/RConn1

== system afe_inv_ttype_psm/afe_abc_inv_psm_mod1/LCL_filter/threephase_vi_measures_stack ==
  Bus Creator : BusCreator  Inputs=6
  Current Sensor : fl_lib/Electrical/Electrical Sensors/Current Sensor
  Current Sensor1 : fl_lib/Electrical/Electrical Sensors/Current Sensor
  Current Sensor2 : fl_lib/Electrical/Electrical Sensors/Current Sensor
  Electrical Reference1 : fl_lib/Electrical/Electrical Elements/Electrical Reference
  Gain : Gain  Gain=1/3
  Gain1 : Gain  Gain=1/hwdata.afe.ubez
  Gain2 : Gain  Gain=1/hwdata.afe.ubez
  Gain3 : Gain  Gain=1/hwdata.afe.ubez
  Gain4 : Gain  Gain=1/hwdata.afe.ibez
  Gain5 : Gain  Gain=1/hwdata.afe.ibez
  Gain6 : Gain  Gain=1/hwdata.afe.ibez
  Selector : Selector  InputPortWidth=6  IndexOptions=Index vector (dialog)  Indices=[1 2 3]  OutputSizes=1
  Selector1 : Selector  InputPortWidth=6  IndexOptions=Index vector (dialog)  Indices=[4 5 6]  OutputSizes=1
  Sum : Sum  Inputs=+++
  Voltage Sensor : fl_lib/Electrical/Electrical Sensors/Voltage Sensor
  Voltage Sensor1 : fl_lib/Electrical/Electrical Sensors/Voltage Sensor
  Voltage Sensor2 : fl_lib/Electrical/Electrical Sensors/Voltage Sensor
  ia_afe : nesl_utility/PS-Simulink Converter  PhysicalDomain=network_engine_domain  SubClassName=ps_output  LeftPortType=input  RightPortType=output  PseudoPeriodic=off  Frequencies=[]  VectorFormat=1-D array  Unit=A  AffineConversion=off
  ib_afe : nesl_utility/PS-Simulink Converter  PhysicalDomain=network_engine_domain  SubClassName=ps_output  LeftPortType=input  RightPortType=output  PseudoPeriodic=off  Frequencies=[]  VectorFormat=1-D array  Unit=A  AffineConversion=off
  ic_afe : nesl_utility/PS-Simulink Converter  PhysicalDomain=network_engine_domain  SubClassName=ps_output  LeftPortType=input  RightPortType=output  PseudoPeriodic=off  Frequencies=[]  VectorFormat=1-D array  Unit=A  AffineConversion=off
  ua_afe : nesl_utility/PS-Simulink Converter  PhysicalDomain=network_engine_domain  SubClassName=ps_output  LeftPortType=input  RightPortType=output  PseudoPeriodic=off  Frequencies=[]  VectorFormat=1-D array  Unit=V  AffineConversion=off
  ub_afe : nesl_utility/PS-Simulink Converter  PhysicalDomain=network_engine_domain  SubClassName=ps_output  LeftPortType=input  RightPortType=output  PseudoPeriodic=off  Frequencies=[]  VectorFormat=1-D array  Unit=V  AffineConversion=off
  uc_afe : nesl_utility/PS-Simulink Converter  PhysicalDomain=network_engine_domain  SubClassName=ps_output  LeftPortType=input  RightPortType=output  PseudoPeriodic=off  Frequencies=[]  VectorFormat=1-D array  Unit=V  AffineConversion=off
  Ua : PMIOPort  Side=Left
  ua : PMIOPort  Port=2  Side=Right
  Ub : PMIOPort  Port=3  Side=Left
  ub : PMIOPort  Port=4  Side=Right
  Uc : PMIOPort  Port=5  Side=Left
  uc : PMIOPort  Port=6  Side=Right
  tag scope: is_abc_pu_mod1=global, iz_afe_pu_mod1=global, vs_abc_pu_mod1=global
  wires:
  Bus Creator/1 -> Selector/1, Selector1/1  "vi_data"
  Selector/1 -> [vs_abc_pu_mod1]
  ib_afe/1 -> Gain4/1  "ib_afe"
  ia_afe/1 -> Gain6/1  "ia_afe"
  ic_afe/1 -> Gain5/1  "ic_afe"
  ua_afe/1 -> Gain1/1  "ua_afe"
  ub_afe/1 -> Gain2/1  "ub_afe"
  uc_afe/1 -> Gain3/1  "uc_afe"
  Selector1/1 -> [is_abc_pu_mod1]
  Sum/1 -> Gain/1
  Gain/1 -> [iz_afe_pu_mod1]
  Gain1/1 -> Bus Creator/1  "ua_afe_pu"
  Gain2/1 -> Bus Creator/2  "ub_afe_pu"
  Gain3/1 -> Bus Creator/3  "uc_afe_pu"
  Gain6/1 -> Sum/1, Bus Creator/4  "ia_afe_pu"
  Gain4/1 -> Sum/2, Bus Creator/5  "ib_afe_pu"
  Gain5/1 -> Bus Creator/6, Sum/3  "ic_afe_pu"
  connections:
  Current Sensor1/LConn1 -- Ub/RConn1 -- Voltage Sensor1/LConn1
  Electrical Reference1/LConn1 -- Voltage Sensor/RConn2 -- Voltage Sensor2/RConn2 -- Voltage Sensor1/RConn2
  Voltage Sensor/RConn1 -- ua_afe/LConn1
  Current Sensor/RConn2 -- ua/RConn1
  Voltage Sensor1/RConn1 -- ub_afe/LConn1
  Voltage Sensor2/LConn1 -- Uc/RConn1 -- Current Sensor2/LConn1
  Current Sensor/LConn1 -- Ua/RConn1 -- Voltage Sensor/LConn1
  Current Sensor1/RConn2 -- ub/RConn1
  Voltage Sensor2/RConn1 -- uc_afe/LConn1
  ib_afe/LConn1 -- Current Sensor1/RConn1
  ia_afe/LConn1 -- Current Sensor/RConn1
  ic_afe/LConn1 -- Current Sensor2/RConn1
  Current Sensor2/RConn2 -- uc/RConn1

== system afe_inv_ttype_psm/afe_abc_inv_psm_mod1/afe/deadtime_generator_for_ttype ==
  gate_cmds_in : Inport
  Bus Creator : BusCreator  Inputs=3
  dead_time_generator_cmos_simulink_phu : Subsystem  mask{ts=glb_time.tc, positive_voltage_rail=15, dead_time=glb_time.dead_time_AFE}
      mask prompts: ts "PT1 tau [s]"; positive_voltage_rail "Positive Voltage Rail [V]"; dead_time "DeadTime [s]"
  dead_time_generator_cmos_simulink_phv : Subsystem  mask{ts=glb_time.tc, positive_voltage_rail=15, dead_time=glb_time.dead_time_AFE}
      mask prompts: ts "PT1 tau [s]"; positive_voltage_rail "Positive Voltage Rail [V]"; dead_time "DeadTime [s]"
  dead_time_generator_cmos_simulink_phw : Subsystem  mask{ts=glb_time.tc, positive_voltage_rail=15, dead_time=glb_time.dead_time_AFE}
      mask prompts: ts "PT1 tau [s]"; positive_voltage_rail "Positive Voltage Rail [V]"; dead_time "DeadTime [s]"
  gate_cmds_out : Outport
  wires:
  Bus Creator/1 -> gate_cmds_out/1  "gate_cmds"
  dead_time_generator_cmos_simulink_phu/1(cmd_gates) -> Bus Creator/1  "gate_cmds_phu"
  gate_cmds_in/1 -> dead_time_generator_cmos_simulink_phu/1(gate_commands), dead_time_generator_cmos_simulink_phw/1(gate_commands), dead_time_generator_cmos_simulink_phv/1(gate_commands)
  dead_time_generator_cmos_simulink_phw/1(cmd_gates) -> Bus Creator/3  "gate_cmds_phw"
  dead_time_generator_cmos_simulink_phv/1(cmd_gates) -> Bus Creator/2  "gate_cmds_phv"

== system afe_inv_ttype_psm/afe_abc_inv_psm_mod1/afe/sv_pwm ==
  duties_uvw : Inport
  Bus Selector2 : BusSelector  OutputSignals=du(k),dv(k),dw(k)
  Constant1 : Constant  Value=afe_pwm_phase_shift_mod1
  modulator1 : Subsystem
  td2tc_1 : TransferFcn  Denominator=[glb_time.tc 1]
  td2tc_2 : TransferFcn  Denominator=[glb_time.tc 1]
  td2tc_3 : TransferFcn  Denominator=[glb_time.tc 1]
  gate_cmds : Outport
  wires:
  modulator1/1(gate_cmds) -> gate_cmds/1
  Constant1/1 -> modulator1/4(phase)
  Bus Selector2/1 -> td2tc_1/1  "<du(k)>"
  Bus Selector2/2 -> td2tc_2/1  "<dv(k)>"
  Bus Selector2/3 -> td2tc_3/1  "<dw(k)>"
  duties_uvw/1 -> Bus Selector2/1
  td2tc_1/1 -> modulator1/1(u)  "du(t)"
  td2tc_3/1 -> modulator1/3(w)  "dw(t)"
  td2tc_2/1 -> modulator1/2(v)  "dv(t)"

== system afe_inv_ttype_psm/afe_abc_inv_psm_mod1/brake/Rbrake ==
  PS-Simulink Converter2 : nesl_utility/PS-Simulink Converter  PhysicalDomain=network_engine_domain  SubClassName=ps_output  LeftPortType=input  RightPortType=output  PseudoPeriodic=off  Frequencies=[]  VectorFormat=1-D array  Unit=degC  AffineConversion=off
  PS-Simulink Converter3 : nesl_utility/PS-Simulink Converter  PhysicalDomain=network_engine_domain  SubClassName=ps_output  LeftPortType=input  RightPortType=output  PseudoPeriodic=off  Frequencies=[]  VectorFormat=1-D array  Unit=W  AffineConversion=off
  Rbrake_thermal : Scope  NumInputPorts=2
      settings: ActiveDisplayYMinimum=-0.01108487622474996  ActiveDisplayYMaximum=0.099763886022749659  DataLoggingVariableName=ScopeData33
  Resistor1 : ee_lib/Passive/Resistor  R=hwdata.afe.Rbrake Ohm  enable_R_tol=ee.enum.toleranceApplication.none  R_tol=5  tol_distribution=ee.enum.toleranceDistribution.uniform  nSigma=4  enable_operating_limits=ee.enum.enable.no  operating_limit_action=ee.enum.passive.reportOpLim.warn  power_rating=1 W  max_working_voltage=100 V  noise_mode=ee.enum.sources.noise.Disabled  Tdevice=25 degC  sample_time=1e-3 s  repeatability=ee.enum.ic.repeatability.notRepeatable  user_seed=0  auto_seed=3499211588  power_derating_T1=70 degC  power_derating_T2=155 degC  operating_temperature_range_vec=[-50, 150] degC  alpha=3.93e-3 1/K  Tmeas=25 degC  thermal_mass=100 J/K  temperature_specify=off  temperature_priority=High  temperature=298.15 K  temperature_nominal_specify=off  temperature_nominal_value=1  temperature_nominal_unit=K
  Tambient : fl_lib/Thermal/Thermal Sources/Temperature Source  temperature=Tambient degC
  Temperature Sensor1 : fl_lib/Thermal/Thermal Sensors/Temperature Sensor  temperature_measure=foundation.enum.MeasurementReference.difference
  To Workspace1 : ToWorkspace  VariableName=RbrakePowerFlow_mod1_sim  SampleTime=glb_time.tc
      settings: MaxDataPoints=glb_time.Nc
  To Workspace10 : ToWorkspace  VariableName=RbrakeTemperature_mod1_sim  SampleTime=glb_time.tc
      settings: MaxDataPoints=glb_time.Nc
  heatsink_C : fl_lib/Thermal/Thermal Elements/Thermal Mass  mass_type=foundation.enum.constant_variable.constant  mass=40 kg  sp_heat=505 J/(K*kg)  mass_min=1e-6 kg  num_ports=foundation.enum.numPorts2.one  m_specify=off  m_priority=High  m=1 kg  m_nominal_specify=off  m_nominal_value=1  m_nominal_unit=kg  T_specify=on  T_priority=High  T=DThs_init+Tambient degC  T_nominal_specify=off  T_nominal_value=1  T_nominal_unit=K  Q_specify=off  Q_priority=High  Q=0 W  Q_nominal_specify=off  Q_nominal_value=1  Q_nominal_unit=W
  power_losses_switch : fl_lib/Thermal/Thermal Sensors/Heat Flow Rate Sensor
  switch_heatsink : fl_lib/Thermal/Thermal Elements/Thermal Resistance  resistance=300/48e3 K/W  T_specify=off  T_priority=High  T=0 deltadegC  T_nominal_specify=off  T_nominal_value=1  T_nominal_unit=K  Q_specify=off  Q_priority=None  Q=0 W  Q_nominal_specify=off  Q_nominal_value=1  Q_nominal_unit=W
  A : PMIOPort  Side=Left
  B : PMIOPort  Port=2  Side=Right
  wires:
  PS-Simulink Converter2/1 -> To Workspace10/1, Rbrake_thermal/1  "RbrakeTemperature"
  PS-Simulink Converter3/1 -> To Workspace1/1, Rbrake_thermal/2  "RbrakePowerFlow"
  connections:
  Resistor1/LConn1 -- A/RConn1
  Resistor1/RConn1 -- B/RConn1
  Tambient/LConn1 -- Temperature Sensor1/RConn1 -- switch_heatsink/RConn1
  Temperature Sensor1/LConn1 -- power_losses_switch/RConn2 -- heatsink_C/LConn1 -- switch_heatsink/LConn1
  Temperature Sensor1/RConn2 -- PS-Simulink Converter2/LConn1
  power_losses_switch/LConn1 -- Resistor1/LConn2
  power_losses_switch/RConn1 -- PS-Simulink Converter3/LConn1

== system afe_inv_ttype_psm/afe_abc_inv_psm_mod1/brake/switch_1 ==
  Capacitor : fl_lib/Electrical/Electrical Elements/Capacitor  c=ideal_switch.Csnubber F  r=ideal_switch.Rsnubber Ohm  g=0 1/Ohm  i_specify=off  i_priority=None  i=0 A  i_nominal_specify=off  i_nominal_value=1  i_nominal_unit=A  v_specify=off  v_priority=None  v=0 V  v_nominal_specify=off  v_nominal_value=1  v_nominal_unit=V  vc_specify=off  vc_priority=High  vc=0 V  vc_nominal_specify=off  vc_nominal_value=1  vc_nominal_unit=V
  Diode : fl_lib/Electrical/Electrical Elements/Diode  Vf=ideal_switch.Vgamma V  Ron=ideal_switch.Rdon_diode Ohm  Goff=1e-8 1/Ohm  i_specify=off  i_priority=None  i=0 A  i_nominal_specify=off  i_nominal_value=1  i_nominal_unit=A  v_specify=off  v_priority=None  v=0 V  v_nominal_specify=off  v_nominal_value=1  v_nominal_unit=V
  C : PMIOPort  Side=Left
  E : PMIOPort  Port=2  Side=Right
  connections:
  Diode/LConn1 -- Capacitor/RConn1 -- E/RConn1
  Diode/RConn1 -- C/RConn1 -- Capacitor/LConn1

== system afe_inv_ttype_psm/afe_abc_inv_psm_mod1/brake/switch_2 ==
  Capacitor : fl_lib/Electrical/Electrical Elements/Capacitor  c=ideal_switch.Csnubber F  r=ideal_switch.Rsnubber Ohm  g=0 1/Ohm  i_specify=off  i_priority=None  i=0 A  i_nominal_specify=off  i_nominal_value=1  i_nominal_unit=A  v_specify=off  v_priority=None  v=0 V  v_nominal_specify=off  v_nominal_value=1  v_nominal_unit=V  vc_specify=off  vc_priority=High  vc=0 V  vc_nominal_specify=off  vc_nominal_value=1  vc_nominal_unit=V
  Diode : fl_lib/Electrical/Electrical Elements/Diode  Vf=ideal_switch.Vgamma V  Ron=ideal_switch.Rdon_diode Ohm  Goff=1e-8 1/Ohm  i_specify=off  i_priority=None  i=0 A  i_nominal_specify=off  i_nominal_value=1  i_nominal_unit=A  v_specify=off  v_priority=None  v=0 V  v_nominal_specify=off  v_nominal_value=1  v_nominal_unit=V
  Switch : fl_lib/Electrical/Electrical Elements/Switch  R_closed=ideal_switch.Rds_on Ohm  G_open=1e-8 1/Ohm  Threshold=7.5  i_specify=off  i_priority=None  i=0 A  i_nominal_specify=off  i_nominal_value=1  i_nominal_unit=A  v_specify=off  v_priority=None  v=0 V  v_nominal_specify=off  v_nominal_value=1  v_nominal_unit=V
  G : PMIOPort  Side=Left
  C : PMIOPort  Port=2  Side=Left
  E : PMIOPort  Port=3  Side=Right
  connections:
  Switch/RConn2 -- C/RConn1 -- Capacitor/LConn1 -- Diode/RConn1
  Switch/RConn1 -- G/RConn1
  Switch/LConn1 -- E/RConn1 -- Capacitor/RConn1 -- Diode/LConn1

== system afe_inv_ttype_psm/afe_abc_inv_psm_mod1/inv_psm_mod1/dclink ==
  Bus Selector : BusSelector  OutputSignals=vdc_pu,udc,udc1,udc2,np_current,udc_p_gnd,udc_n_gnd,udc_centertap_gnd,Cdc1_current,Cdc2_current,udc1_pu,udc2_pu
  dclink : dclink_for_three_levels/dclink  Cdc1_m=hwdata.afe.CFi1  Cdc2_m=hwdata.afe.CFi2  Rudc_measure=1e6  Vdc_scale=hwdata.afe.udc_nom  Vdc1_m_init=hwdata.afe.udc_nom/2  Vdc2_m_init=hwdata.afe.udc_nom/2
  Udc(+) : PMIOPort  Side=Left
  Np : PMIOPort  Port=2  Side=Left
  Udc(-) : PMIOPort  Port=3  Side=Left
  udc(+) : PMIOPort  Port=4  Side=Right
  np : PMIOPort  Port=5  Side=Right
  udc(-) : PMIOPort  Port=6  Side=Right
  tag scope: Cdc1_current=scoped, Cdc2_current=scoped, np_current=scoped, udc1=scoped, udc1_inv_mod1=global, udc1_pu=scoped, udc1_pu_inv_mod1=global, udc2=scoped, udc2_inv_mod1=global, udc2_pu=scoped, udc2_pu_inv_mod1=global, udc=scoped, udc_centertap_gnd=scoped, udc_n_gnd=scoped, udc_p_gnd=scoped, vdc_pu=scoped, vdc_pu_inv_mod1=global
  wires:
  Bus Selector/6 -> [udc_p_gnd]  "<udc_p_gnd>"
  Bus Selector/8 -> [udc_centertap_gnd]  "<udc_centertap_gnd>"
  Bus Selector/2 -> [udc]  "<udc>"
  Bus Selector/7 -> [udc_n_gnd]  "<udc_n_gnd>"
  dclink/1 -> Bus Selector/1
  Bus Selector/4 -> [udc2]  "<udc2>"
  Bus Selector/9 -> [Cdc1_current]  "<Cdc1_current>"
  Bus Selector/5 -> [np_current]  "<np_current>"
  Bus Selector/3 -> [udc1]  "<udc1>"
  Bus Selector/10 -> [Cdc2_current]  "<Cdc2_current>"
  [vdc_pu] -> [vdc_pu_inv_mod1]
  Bus Selector/12 -> [udc2_pu]  "<udc2_pu>"
  Bus Selector/11 -> [udc1_pu]  "<udc1_pu>"
  [udc1_pu] -> [udc1_pu_inv_mod1]
  [udc2_pu] -> [udc2_pu_inv_mod1]
  [udc2] -> [udc2_inv_mod1]
  [udc1] -> [udc1_inv_mod1]
  Bus Selector/1 -> [vdc_pu]  "<vdc_pu>"
  connections:
  dclink/RConn3 -- Udc(-)/RConn1
  dclink/RConn1 -- Udc(+)/RConn1
  udc(+)/RConn1 -- dclink/LConn1
  np/RConn1 -- dclink/LConn2
  udc(-)/RConn1 -- dclink/LConn3
  Np/RConn1 -- dclink/RConn2

== system afe_inv_ttype_psm/afe_abc_inv_psm_mod1/inv_psm_mod1/inverter ==
  gate_cmds_uvw : Inport
  Bus Creator : BusCreator  Inputs=2
  Current Sensor : fl_lib/Electrical/Electrical Sensors/Current Sensor
  PS-Simulink Converter1 : nesl_utility/PS-Simulink Converter  PhysicalDomain=network_engine_domain  SubClassName=ps_output  LeftPortType=input  RightPortType=output  PseudoPeriodic=off  Frequencies=[]  VectorFormat=1-D array  Unit=A  AffineConversion=on
  PS-Simulink Converter4 : nesl_utility/PS-Simulink Converter  PhysicalDomain=network_engine_domain  SubClassName=ps_output  LeftPortType=input  RightPortType=output  PseudoPeriodic=off  Frequencies=[]  VectorFormat=1-D array  Unit=V  AffineConversion=on
  To Workspace : ToWorkspace  VariableName=idc_sim_mod1  SampleTime=glb_time.tc
      settings: MaxDataPoints=glb_time.Nc
  To Workspace1 : ToWorkspace  VariableName=udc_sim_mod1  SampleTime=glb_time.tc
      settings: MaxDataPoints=glb_time.Nc
  Transfer Fcn : TransferFcn  Denominator=[1e-2 1]
  Voltage Sensor : fl_lib/Electrical/Electrical Sensors/Voltage Sensor
  deadtime_generator_for_ttype : Subsystem
  idc/udc : Scope  NumInputPorts=2
      settings: SampleTime=glb_time.tc  ActiveDisplayYMinimum=-35.22322330009689  ActiveDisplayYMaximum=317.00900970087207  DataLoggingVariableName=ScopeData8
  ideal_switch_based_three_level_inverter_ttype : three_phase_three_level_ttype_inverter_ideal_switch_based_model/ideal_switch_based_three_level_inverter_ttype  Vth=5.5  Ron=1.5e-3  Vdon_diode=2  Rdon_diode=0.15e-3  Csnubber=10e-9  Rsnubber=2200
  timer : Subsystem  mask{f=glb_time.fPWM_INV, m_up=0.98, m_low=0.02, dead_time=glb_time.dead_time_INV, pos_cmd_gate=15, neg_cmd_gate=-10, polarity=1, tc=glb_time.tc, double_sampling=glb_time.TRGO_INV_double_update}
      mask prompts: f "Frequency (Hz)"; m_up "Max Input Modulation Value"; m_low "Min Input Modulation Value"; dead_time "Dead Time (s)"; pos_cmd_gate "Positive Gate Voltage (V)"; neg_cmd_gate "Negative Gate Voltage (V)"; polarity "Polarity (pu)"; tc "Sampling time"
  udc_scope : Scope  NumInputPorts=3
      settings: ActiveDisplayYMinimum=0.97742270953395249  ActiveDisplayYMaximum=0.98060545699905033  DataLoggingVariableName=ScopeData6
  Udc(+) : PMIOPort  Side=Right
  np : PMIOPort  Port=2  Side=Right
  Udc(-) : PMIOPort  Port=3  Side=Right
  us_u : PMIOPort  Port=4  Side=Left
  us_v : PMIOPort  Port=5  Side=Left
  us_w : PMIOPort  Port=6  Side=Left
  tag scope: TRGO_inv_module_1=global
  wires:
  PS-Simulink Converter4/1 -> To Workspace1/1, idc/udc/2  "udc"
  PS-Simulink Converter1/1 -> Transfer Fcn/1  "idc"
  Transfer Fcn/1 -> idc/udc/1, To Workspace/1  "idc_flt"
  [vdc_pu] -> udc_scope/2  "udc_pu"
  [udc] -> udc_scope/1  "udc"
  [time_inv_module_1] -> timer/1(time_source)
  timer/1(TRGO) -> [TRGO_inv_module_1]
  gate_cmds_uvw/1 -> deadtime_generator_for_ttype/1(gate_cmds_in)
  deadtime_generator_for_ttype/1(gate_cmds_out) -> ideal_switch_based_three_level_inverter_ttype/1
  [udc1] -> Bus Creator/1  "udc_1"
  [udc2] -> Bus Creator/2  "udc_2"
  Bus Creator/1 -> udc_scope/3
  connections:
  PS-Simulink Converter4/LConn1 -- Voltage Sensor/RConn1
  ideal_switch_based_three_level_inverter_ttype/LConn1 -- us_u/RConn1
  ideal_switch_based_three_level_inverter_ttype/LConn2 -- us_v/RConn1
  ideal_switch_based_three_level_inverter_ttype/LConn3 -- us_w/RConn1
  Voltage Sensor/RConn2 -- ideal_switch_based_three_level_inverter_ttype/RConn3 -- Udc(-)/RConn1
  Current Sensor/LConn1 -- Udc(+)/RConn1
  Voltage Sensor/LConn1 -- ideal_switch_based_three_level_inverter_ttype/RConn1 -- Current Sensor/RConn2
  PS-Simulink Converter1/LConn1 -- Current Sensor/RConn1
  np/RConn1 -- ideal_switch_based_three_level_inverter_ttype/RConn2

== system afe_inv_ttype_psm/afe_abc_inv_psm_mod1/inv_psm_mod1/inverter_ctrl ==
  inverter_control : Subsystem
  cmd_gates : Outport
  tag scope: local_time_corr_inv1=global, master_torque_ref=global
  wires:
  [is_uvw_pu_mod1] -> inverter_control/1(is_uvw)
  [TRGO_inv_module_1] -> inverter_control/Trigger
  inverter_control/1(cmd_gates) -> cmd_gates/1
  [time_inv_module_1] -> inverter_control/4(local_time)
  [time_master] -> inverter_control/5(master_time)
  inverter_control/2(local_time_corr) -> [local_time_corr_inv1]
  inverter_control/3(master_torque_ref) -> [master_torque_ref]
  [phase_elec_psm] -> inverter_control/6(theta_elec_psm)
  [omega_elec_psm] -> inverter_control/7(omega_elec_psm)
  [udc1_pu] -> inverter_control/2(udc1_pu)  "udc1_pu"
  [udc2_pu] -> inverter_control/3(udc2_pu)  "udc2_pu"

== system afe_inv_ttype_psm/afe_abc_inv_psm_mod1/inv_psm_mod1/inverter_output_filter ==
  Inductor : fl_lib/Electrical/Electrical Elements/Inductor  l=1e-6 H  r=0 Ohm  g=1e-9 1/Ohm  i_specify=off  i_priority=None  i=0 A  i_nominal_specify=off  i_nominal_value=1  i_nominal_unit=A  v_specify=off  v_priority=None  v=0 V  v_nominal_specify=off  v_nominal_value=1  v_nominal_unit=V  i_L_specify=off  i_L_priority=High  i_L=0 A  i_L_nominal_specify=off  i_L_nominal_value=1  i_L_nominal_unit=A
  Inductor1 : fl_lib/Electrical/Electrical Elements/Inductor  l=1e-6 H  r=0 Ohm  g=1e-9 1/Ohm  i_specify=off  i_priority=None  i=0 A  i_nominal_specify=off  i_nominal_value=1  i_nominal_unit=A  v_specify=off  v_priority=None  v=0 V  v_nominal_specify=off  v_nominal_value=1  v_nominal_unit=V  i_L_specify=off  i_L_priority=High  i_L=0 A  i_L_nominal_specify=off  i_L_nominal_value=1  i_L_nominal_unit=A
  Inductor2 : fl_lib/Electrical/Electrical Elements/Inductor  l=1e-6 H  r=0 Ohm  g=1e-9 1/Ohm  i_specify=off  i_priority=None  i=0 A  i_nominal_specify=off  i_nominal_value=1  i_nominal_unit=A  v_specify=off  v_priority=None  v=0 V  v_nominal_specify=off  v_nominal_value=1  v_nominal_unit=V  i_L_specify=off  i_L_priority=High  i_L=0 A  i_L_nominal_specify=off  i_L_nominal_value=1  i_L_nominal_unit=A
  threephase inductor : threephase_inductor_lib/threephase inductor  Lp=hwdata.inv.LFi H  L0=hwdata.inv.LFi_cm H  Rp=hwdata.inv.RLFi Ohm  R0=hwdata.inv.RLFi_cm Ohm  Lls=5e-6 H  uu_1_specify=off  uu_1_priority=None  uu_1=0 V  uu_1_nominal_specify=off  uu_1_nominal_value=1  uu_1_nominal_unit=V  uv_1_specify=off  uv_1_priority=None  uv_1=0 V  uv_1_nominal_specify=off  uv_1_nominal_value=1  uv_1_nominal_unit=V  uw_1_specify=off  uw_1_priority=None  uw_1=0 V  uw_1_nominal_specify=off  uw_1_nominal_value=1  uw_1_nominal_unit=V  uu_2_specify=off  uu_2_priority=None  uu_2=0 V  uu_2_nominal_specify=off  uu_2_nominal_value=1  uu_2_nominal_unit=V  uv_2_specify=off  uv_2_priority=None  uv_2=0 V  uv_2_nominal_specify=off  uv_2_nominal_value=1  uv_2_nominal_unit=V  uw_2_specify=off  uw_2_priority=None  uw_2=0 V  uw_2_nominal_specify=off  uw_2_nominal_value=1  uw_2_nominal_unit=V  iu_specify=off  iu_priority=None  iu=0 A  iu_nominal_specify=off  iu_nominal_value=1  iu_nominal_unit=A  iv_specify=off  iv_priority=None  iv=0 A  iv_nominal_specify=off  iv_nominal_value=1  iv_nominal_unit=A  iw_specify=off  iw_priority=None  iw=0 A  iw_nominal_specify=off  iw_nominal_value=1  iw_nominal_unit=A
  threephase_vi_measures_stack : Subsystem
  us_u : PMIOPort  Side=Left
  uu : PMIOPort  Port=2  Side=Right
  us_v : PMIOPort  Port=3  Side=Left
  uv : PMIOPort  Port=4  Side=Right
  us_w : PMIOPort  Port=5  Side=Left
  uw : PMIOPort  Port=6  Side=Right
  connections:
  threephase_vi_measures_stack/LConn1 -- us_u/RConn1
  threephase_vi_measures_stack/LConn2 -- us_v/RConn1
  threephase_vi_measures_stack/LConn3 -- us_w/RConn1
  threephase inductor/LConn1 -- threephase_vi_measures_stack/RConn1
  threephase inductor/LConn2 -- threephase_vi_measures_stack/RConn2
  threephase inductor/LConn3 -- threephase_vi_measures_stack/RConn3
  threephase inductor/RConn1 -- Inductor/LConn1
  threephase inductor/RConn2 -- Inductor1/LConn1
  threephase inductor/RConn3 -- Inductor2/LConn1
  Inductor/RConn1 -- uu/RConn1
  Inductor1/RConn1 -- uv/RConn1
  Inductor2/RConn1 -- uw/RConn1
